simulink library "lib_DC_BUCK"  (R2026a)
settings: Solver=VariableStepAuto
undefined symbols (not defined in the file): block_buses, block_idx, block_toM, buses_lf, op_DCBUCK
settings Model: Creator=atomas  LastModifiedBy=atomas

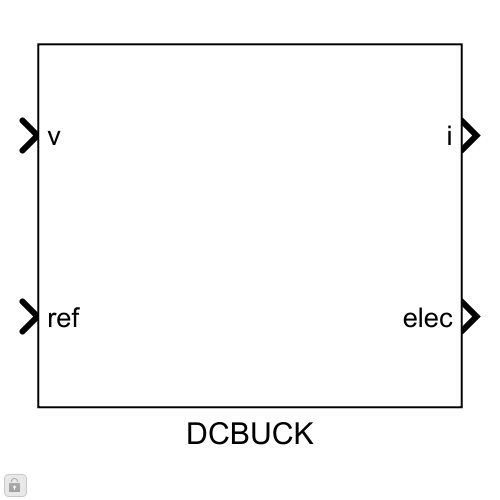
[thumbnail: Simulink's stored preview of the top-level diagram]
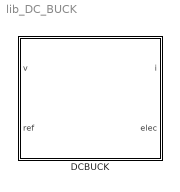
== system lib_DC_BUCK ==
  DCBUCK : Subsystem
      mask init:
      | [block_buses, block_Pg, block_toM, block_idx] = mask_init_DCBUCK(gcb);

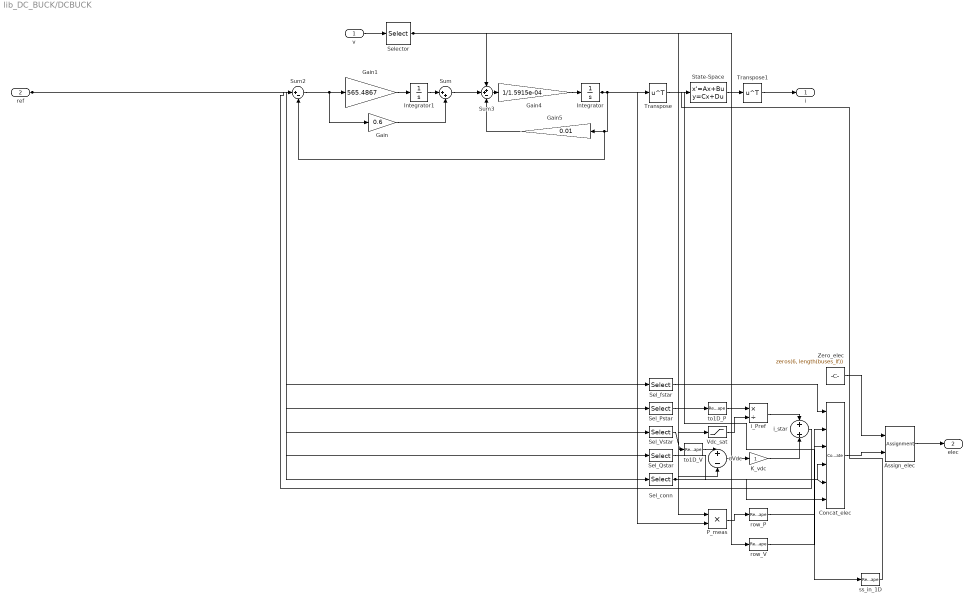
== system lib_DC_BUCK/DCBUCK ==
  v : Inport
  ref : Inport  Port=2
  Assign_elec : Assignment  NumberOfDimensions=2  DiagnosticForDimensions=Warning  IndexOptions=Assign all,Index vector (dialog)  Indices=1,block_idx  OutputSizes=1
  Concat_elec : Concatenate  NumInputs=6  Mode=Multidimensional array
  Gain : Gain  Gain=0.6
  Gain1 : Gain  Gain=565.4867
  Gain4 : Gain  Gain=1/1.5915e-04
  Gain5 : Gain  Gain=0.01
  Integrator : Integrator  InitialCondition=op_DCBUCK.Integrator
  Integrator1 : Integrator  InitialCondition=op_DCBUCK.Integrator1
  K_vdc : Gain
  P_meas : Product  Inputs=**
  Sel_Pstar : Selector  NumberOfDimensions=2  InputPortWidth=3  IndexOptions=Index vector (dialog),Index vector (dialog)  Indices=2,block_idx  OutputSizes=1
  Sel_Qstar : Selector  NumberOfDimensions=2  InputPortWidth=3  IndexOptions=Index vector (dialog),Index vector (dialog)  Indices=4,block_idx  OutputSizes=1
  Sel_Vstar : Selector  NumberOfDimensions=2  InputPortWidth=3  IndexOptions=Index vector (dialog),Index vector (dialog)  Indices=3,block_idx  OutputSizes=1
  Sel_conn : Selector  NumberOfDimensions=2  InputPortWidth=3  IndexOptions=Index vector (dialog),Index vector (dialog)  Indices=5,block_idx  OutputSizes=1
  Sel_fstar : Selector  NumberOfDimensions=2  InputPortWidth=3  IndexOptions=Index vector (dialog),Index vector (dialog)  Indices=1,block_idx  OutputSizes=1
  Selector : Selector  InputPortWidth=DC.Nbuses  IndexOptions=Index vector (dialog)  Indices=block_buses  OutputSizes=1
  State-Space : StateSpace  A=[]  B=[]  C=[]  D=block_toM  InitialCondition=0  ParameterTunability=Optimized
  Sum : Sum  Inputs=|++
  Sum2 : Sum  Inputs=|+-
  Sum3 : Sum  Inputs=++-
  Transpose : Math  Operator=transpose
  Transpose1 : Math  Operator=transpose
  Vdc_sat : Saturate  UpperLimit=inf  LowerLimit=0.1
  Zero_elec : Constant  Value=zeros(6, length(buses_lf))
  dVdc : Sum  Inputs=+-
  i_Pref : Product  Inputs=*/
  i_star : Sum
  row_P : Reshape  OutputDimensionality=Customize  OutputDimensions=[1, length(block_buses)]
  row_V : Reshape  OutputDimensionality=Customize  OutputDimensions=[1, length(block_buses)]
  ss_in_1D : Reshape
  to1D_P : Reshape
  to1D_V : Reshape
  i : Outport
  elec : Outport  Port=2
  wires:
  Gain5/1 -> Sum3/3
  Selector/1 -> Sum3/1, Vdc_sat/1, dVdc/2, P_meas/1, row_V/1
  v/1 -> Selector/1
  Sum3/1 -> Gain4/1
  Transpose1/1 -> i/1
  Sum2/1 -> Gain/1, Gain1/1
  Gain4/1 -> Integrator/1
  Integrator1/1 -> Sum/1
  Gain/1 -> Sum/2
  Sum/1 -> Sum3/2
  Gain1/1 -> Integrator1/1
  Integrator/1 -> Transpose/1, Gain5/1, Sum2/2, P_meas/2
  State-Space/1 -> Transpose1/1
  ref/1 -> Sel_fstar/1, Sel_Pstar/1, Sel_Vstar/1, Sel_Qstar/1, Sel_conn/1
  Vdc_sat/1 -> i_Pref/2
  dVdc/1 -> K_vdc/1
  i_Pref/1 -> i_star/1
  K_vdc/1 -> i_star/2
  i_star/1 -> Sum2/1
  Sel_fstar/1 -> Concat_elec/1
  Sel_Qstar/1 -> Concat_elec/4
  Sel_conn/1 -> Concat_elec/5, Concat_elec/6
  Zero_elec/1 -> Assign_elec/1
  Concat_elec/1 -> Assign_elec/2
  Assign_elec/1 -> elec/1
  Sel_Pstar/1 -> to1D_P/1
  to1D_P/1 -> i_Pref/1
  Sel_Vstar/1 -> to1D_V/1
  to1D_V/1 -> dVdc/1
  P_meas/1 -> row_P/1
  row_P/1 -> Concat_elec/2
  row_V/1 -> Concat_elec/3
  Transpose/1 -> ss_in_1D/1
  ss_in_1D/1 -> State-Space/1
